simulink model "microgrid_top_fixed"  (R2025a)
settings: Solver=FixedStepDiscrete  StartTime=0.0  StopTime=T_stop  FixedStep=Ts  RelTol=1e-3
InitFcn:
  | init_microgrid;
undefined symbols (not defined in the file): C_dc, C_sc, d, DiscIntNeverNeededParam, dt, Emax, eta_inv, G_day, Ion, Ki_ib, Ki_isc, Ki_v, Kp_ib, Kp_isc, Kp_v, Lithium, LOAD_SIGN, Pbmax, Pmax, prof, Pscale, Q_sim_Ah, R_bat, sig, SoC0, SoC_min, T_amb_day, t_day, t_hour, tau_lpf, Tc, th1, th1_act, th2, th2_act, Ts, Ts_ems, Ts_fc, V_bat_nom, V_dc_ref, V_sc_nom
libraries: spsSeriesRLCBranchLib x9, slpidlib x5, spsVoltageMeasurementLib x5, spsIdealSwitchLib x5, spsIGBTDiodeLib x4, spsCurrentMeasurementLib x3, simulink x3, spsParallelRLCLoadLib x3, spsPWMGeneratorDCDCLib x2, spsDiodeLib x2, spsPVArrayLib x2, spsBatteryLib x1
(part 2 of 2)

== matlab function microgrid_top_fixed/PV Array (2 x 19.2 kW)/PV Generation 2/PandO ==
  data: Vpv input; D output; Ipv input
function D = PandO(Vpv, Ipv)
% P&O MPPT with night parking, for a boost converter on a 400 V bus.
% Vpv = (1 - D) * Vbus, so lowering D raises the PV voltage.
persistent Vold Pold Dold
if isempty(Vold), Vold = 0; Pold = 0; Dold = 0.42; end
dD = 0.002;  Pmin = 150;  D_park = 0.42;
P  = Vpv*Ipv;  dV = Vpv - Vold;  dP = P - Pold;
if P < Pmin          % night or very weak light: park near 0.8*Voc
    D = D_park;
elseif dP == 0
    D = Dold;
elseif dP*dV > 0     % left of MPP: raise Vpv by lowering D
    D = Dold - dD;
else                 % right of MPP: lower Vpv by raising D
    D = Dold + dD;
end
% Voltage window: Vpv command 160-256 V (D 0.36-0.60). Covers every MPP
% of the day (~195-245 V) but never asks for more than Voc (~255+ V),
% so P&O cannot drift to open circuit when irradiance rises at sunrise.
D = min(max(D, 0.36), 0.60);
Vold = Vpv; Pold = P; Dold = D;

== matlab function microgrid_top_fixed/EMS (LPF power split)/BESS/MATLAB Function ==
  data: Pbat_base input; Pbat_adaptive output; SOC_Bat input
function Pbat_adaptive = fcn(Pbat_base, SOC_Bat)

if SOC_Bat < 30 && Pbat_base > 0
    Pbat_adaptive = 0.2 * Pbat_base;

elseif SOC_Bat > 90 && Pbat_base < 0
    Pbat_adaptive = 0.2 * Pbat_base;

else
    Pbat_adaptive = Pbat_base;
end

== stateflow chart microgrid_top_fixed/Load Manager (adaptive shedding)/Load Manager ==
  settings: updateMethod=DISCRETE  sampleTime=Ts_ems
  state L0_Normal
    en:L=0;
    outage_flag = 0;
  state L1_ShedDeferrable
    en:L=1;
    outage_flag = 0;
  state L2_CriticalOnly
    en:L=2;
    outage_flag = 0;
  state L3_Outage
    en: L = 3;
    outage_flag = 1;
  L1_ShedDeferrable -> L2_CriticalOnly [order 1] : [SoC < th2_act]
  L0_Normal -> L1_ShedDeferrable : [SoC < th1_act || (SoC < th1_act + 0.05 && dSoC_dt < -0.15)]
  L2_CriticalOnly -> L3_Outage [order 2] : [SoC <= SoC_min || P_def > 22]
  (default) -> L0_Normal
  L3_Outage -> L0_Normal : [SoC > SoC_min + 0.10 && P_def <= 10]
  L1_ShedDeferrable -> L0_Normal [order 2] : [SoC>th1_act+d]
  L2_CriticalOnly -> L1_ShedDeferrable [order 1] : [SoC>th2_act+d]
  data: SoC input; L output; th1 parameter; th2 parameter; d parameter; dSoC_dt input; P_def input; SoC_min parameter; outage_flag output; th2_act parameter; th1_act parameter

== matlab function microgrid_top_fixed/PV Array (2 x 19.2 kW)/PV Generation/PandO ==
  data: Vpv input; D output; Ipv input
function D = PandO(Vpv, Ipv)
% P&O MPPT with night parking, for a boost converter on a 400 V bus.
% Vpv = (1 - D) * Vbus, so lowering D raises the PV voltage.
persistent Vold Pold Dold
if isempty(Vold), Vold = 0; Pold = 0; Dold = 0.42; end
dD = 0.002;  Pmin = 150;  D_park = 0.42;
P  = Vpv*Ipv;  dV = Vpv - Vold;  dP = P - Pold;
if P < Pmin          % night or very weak light: park near 0.8*Voc
    D = D_park;
elseif dP == 0
    D = Dold;
elseif dP*dV > 0     % left of MPP: raise Vpv by lowering D
    D = Dold - dD;
else                 % right of MPP: lower Vpv by raising D
    D = Dold + dD;
end
% Voltage window: Vpv command 160-256 V (D 0.36-0.60). Covers every MPP
% of the day (~195-245 V) but never asks for more than Voc (~255+ V),
% so P&O cannot drift to open circuit when irradiance rises at sunrise.
D = min(max(D, 0.36), 0.60);
Vold = Vpv; Pold = P; Dold = D;
